simulink model "fw_can2_codec"  (R2026b)
settings: Solver=VariableStepAuto
undefined symbols (not defined in the file or in its folder): P, Ts
libraries: simulink x1
settings Model: Creator=aomar  LastModifiedBy=aomar

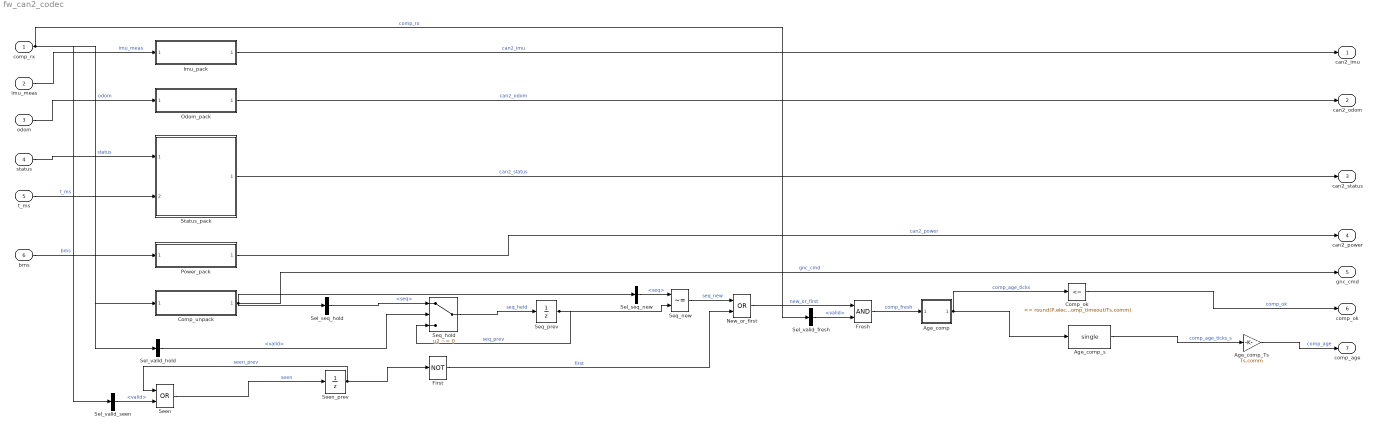
== system fw_can2_codec ==
  comp_rx : Inport  OutDataTypeStr=Bus: Bus_CanFrame64  SampleTime=Ts.comm
  imu_meas : Inport  Port=2  OutDataTypeStr=Bus: Bus_ImuMeas  SampleTime=Ts.imu
  odom : Inport  Port=3  OutDataTypeStr=Bus: Bus_OdomMeas  SampleTime=Ts.ctrl
  status : Inport  Port=4  OutDataTypeStr=Bus: Bus_McuStatus  SampleTime=Ts.comm
  t_ms : Inport  Port=5  OutDataTypeStr=uint32  SampleTime=Ts.comm
  bms : Inport  Port=6  OutDataTypeStr=Bus: Bus_BmsStatus  SampleTime=Ts.hk
  Age_comp : Subsystem
  Age_comp_Ts : Gain  Gain=Ts.comm
  Age_comp_s : DataTypeConversion  OutDataTypeStr=single  RndMeth=Round
  Comp_ok : simulink/Logic and Bit Operations/Compare To Constant  relop=<=  const=round(P.electronics.safety.comp_timeout/Ts.comm)  OutDataTypeStr=boolean
  Comp_unpack : Subsystem  ReferencedSubsystem=can2_comp_cmd_unpack
  First : Logic  Operator=NOT  Inputs=1  AllPortsSameDT=off  OutDataTypeStr=boolean
  Fresh : Logic  AllPortsSameDT=off  OutDataTypeStr=boolean
  Imu_pack : Subsystem  ReferencedSubsystem=can2_mcu_imu_pack
  New_or_first : Logic  Operator=OR  AllPortsSameDT=off  OutDataTypeStr=boolean
  Odom_pack : Subsystem  ReferencedSubsystem=can2_mcu_odom_pack
  Power_pack : Subsystem  ReferencedSubsystem=can2_mcu_power_pack
  Seen : Logic  Operator=OR  AllPortsSameDT=off  OutDataTypeStr=boolean
  Seen_prev : UnitDelay  InitialCondition=false  SampleTime=-1
  Sel_seq_hold : BusSelector  OutputSignals=seq
  Sel_seq_new : BusSelector  OutputSignals=seq
  Sel_valid_fresh : BusSelector  OutputSignals=valid
  Sel_valid_hold : BusSelector  OutputSignals=valid
  Sel_valid_seen : BusSelector  OutputSignals=valid
  Seq_hold : Switch  Criteria=u2 ~= 0  SaturateOnIntegerOverflow=off  InputSameDT=off
  Seq_new : RelationalOperator  Operator=~=  OutDataTypeStr=boolean  RndMeth=Simplest  InputSameDT=off
  Seq_prev : UnitDelay  SampleTime=-1
  Status_pack : Subsystem  ReferencedSubsystem=can2_mcu_status_pack
  can2_imu : Outport  OutDataTypeStr=Bus: Bus_CanFrame64
  can2_odom : Outport  Port=2  OutDataTypeStr=Bus: Bus_CanFrame64
  can2_status : Outport  Port=3  OutDataTypeStr=Bus: Bus_CanFrame64
  can2_power : Outport  Port=4  OutDataTypeStr=Bus: Bus_CanFrame64
  gnc_cmd : Outport  Port=5  OutDataTypeStr=Bus: Bus_GncCmd
  comp_ok : Outport  Port=6  OutDataTypeStr=boolean
  comp_age : Outport  Port=7  OutDataTypeStr=single
  wires:
  comp_rx/1 -> Sel_valid_seen/1, Sel_valid_hold/1, Sel_valid_fresh/1, Comp_unpack/1  "comp_rx"
  imu_meas/1 -> Imu_pack/1  "imu_meas"
  odom/1 -> Odom_pack/1  "odom"
  status/1 -> Status_pack/1  "status"
  t_ms/1 -> Status_pack/2  "t_ms"
  bms/1 -> Power_pack/1  "bms"
  Sel_valid_seen/1 -> Seen/2  "<valid>"
  Sel_valid_hold/1 -> Seq_hold/2  "<valid>"
  Seen/1 -> Seen_prev/1  "seen"
  Imu_pack/1 -> can2_imu/1  "can2_imu"
  Odom_pack/1 -> can2_odom/1  "can2_odom"
  Status_pack/1 -> can2_status/1  "can2_status"
  Power_pack/1 -> can2_power/1  "can2_power"
  Comp_unpack/1 -> gnc_cmd/1, Sel_seq_new/1, Sel_seq_hold/1  "gnc_cmd"
  Sel_seq_hold/1 -> Seq_hold/1  "<seq>"
  Seen_prev/1 -> First/1, Seen/1  "seen_prev"
  First/1 -> New_or_first/2  "first"
  Seq_hold/1 -> Seq_prev/1  "seq_held"
  Seq_prev/1 -> Seq_hold/3, Seq_new/2  "seq_prev"
  Sel_seq_new/1 -> Seq_new/1  "<seq>"
  Seq_new/1 -> New_or_first/1  "seq_new"
  New_or_first/1 -> Fresh/1  "new_or_first"
  Sel_valid_fresh/1 -> Fresh/2  "<valid>"
  Fresh/1 -> Age_comp/1(fresh)  "comp_fresh"
  Age_comp/1(ticks) -> Age_comp_s/1, Comp_ok/1  "comp_age_ticks"
  Comp_ok/1 -> comp_ok/1  "comp_ok"
  Age_comp_s/1 -> Age_comp_Ts/1  "comp_age_ticks_s"
  Age_comp_Ts/1 -> comp_age/1  "comp_age"

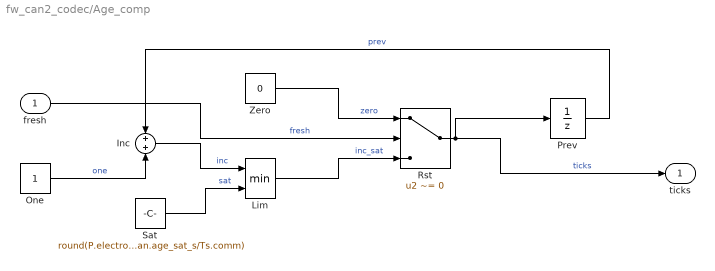
== system fw_can2_codec/Age_comp ==
  fresh : Inport
  Inc : Sum  OutDataTypeStr=uint16  SaturateOnIntegerOverflow=on
  Lim : MinMax  Inputs=2
  One : Constant  OutDataTypeStr=uint16  SampleTime=-1
  Prev : UnitDelay  InitialCondition=round(P.electronics.can.age_sat_s/Ts.comm)  SampleTime=-1
  Rst : Switch  Criteria=u2 ~= 0  SaturateOnIntegerOverflow=off  InputSameDT=off
  Sat : Constant  Value=round(P.electronics.can.age_sat_s/Ts.comm)  OutDataTypeStr=uint16  SampleTime=-1
  Zero : Constant  Value=0  OutDataTypeStr=uint16  SampleTime=-1
  ticks : Outport
  wires:
  fresh/1 -> Rst/2  "fresh"
  One/1 -> Inc/2  "one"
  Inc/1 -> Lim/1  "inc"
  Sat/1 -> Lim/2  "sat"
  Zero/1 -> Rst/1  "zero"
  Lim/1 -> Rst/3  "inc_sat"
  Rst/1 -> ticks/1, Prev/1  "ticks"
  Prev/1 -> Inc/1  "prev"
